simulink model "MPC_Controlled_Booster"  (R2024a)
settings: Solver=VariableStepAuto  StartTime=0  StopTime=1  RelTol=1e-3
values from neighbouring files (symbols this model uses):
  C = (Ioutmax * (1 - (Vin / Vref))) / (fs * delvout)    (= 0.00434027777778)    [RLC_For_MPC.m]
  L = (Vin * (Vref - Vin)) / (delIL * fs * Vref)    (= 0.00144)    [RLC_For_MPC.m]
  R = Vref / Ioutmax    (= 1.152)    [RLC_For_MPC.m]
  Vin = 12    [RLC_For_MPC.m]
libraries: spsSeriesRLCBranchLib x3, spsCurrentMeasurementLib x2, spsVoltageMeasurementLib x2, spsDCVoltageSourceLib x1, spsDiodeLib x1, spsIGBTLib x1, spsPWMGeneratorDCDCLib x1, sps_lib x1
settings Model: Creator=Razowan  LastModifiedBy=Razowan
settings DataIOCC: ReturnWorkspaceOutputs=off

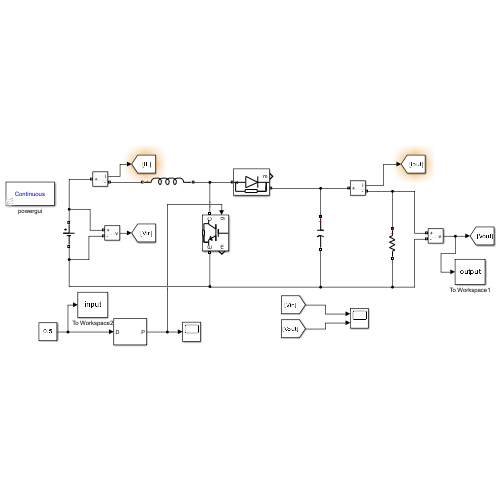
[thumbnail: Simulink's stored preview of the top-level diagram]
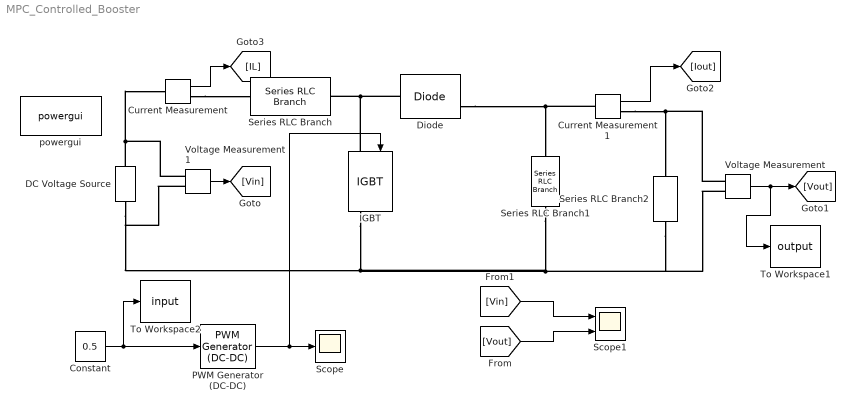
== system MPC_Controlled_Booster ==
  Constant : Constant  Value=0.5
  Current Measurement : spsCurrentMeasurementLib/Current Measurement  PhasorSimulation=off  OutputType=Complex  PSBequivalent=0
  Current Measurement1 : spsCurrentMeasurementLib/Current Measurement  PhasorSimulation=off  OutputType=Complex  PSBequivalent=0
  DC Voltage Source : spsDCVoltageSourceLib/DC Voltage Source  Amplitude=Vin  Measurements=None
  Diode : spsDiodeLib/Diode  Ron=0.001  Lon=0  Vf=0.8  IC=0  UseSnubber=0  Rs=500  Cs=250e-9  Measurements=on
  IGBT : spsIGBTLib/IGBT  Ron=0.001  Lon=0  Vf=1  Tf=1e-6  Tt=2e-6  IC=0  Rs=1e5  Cs=inf  Measurements=on
  PWM Generator (DC-DC) : spsPWMGeneratorDCDCLib/PWM Generator (DC-DC)  Fsw=10000  Ts=0
  Scope : Scope
  Scope1 : Scope  NumInputPorts=2
  Series RLC Branch : spsSeriesRLCBranchLib/Series RLC Branch  LConnTagsString=__new0  RConnTagsString=__new0  BranchType=L  Resistance=1  Inductance=L  SetiL0=off  InitialCurrent=0  Capacitance=1e-6  Setx0=off  InitialVoltage=0  Measurements=None
  Series RLC Branch1 : spsSeriesRLCBranchLib/Series RLC Branch  LConnTagsString=__new0  RConnTagsString=__new0  BranchType=C  Resistance=1  Inductance=L  SetiL0=off  InitialCurrent=0  Capacitance=C  Setx0=off  InitialVoltage=0  Measurements=None
  Series RLC Branch2 : spsSeriesRLCBranchLib/Series RLC Branch  LConnTagsString=__new0  RConnTagsString=__new0  BranchType=R  Resistance=R  Inductance=L  SetiL0=off  InitialCurrent=0  Capacitance=1e-6  Setx0=off  InitialVoltage=0  Measurements=None
  To Workspace1 : ToWorkspace  VariableName=output  SampleTime=0.00001
      settings: Save2DSignal=2-D array (concatenate along first dimension)
  To Workspace2 : ToWorkspace  VariableName=input  SampleTime=0.00001
      settings: Save2DSignal=2-D array (concatenate along first dimension)
  Voltage Measurement : spsVoltageMeasurementLib/Voltage Measurement  PhasorSimulation=off  OutputType=Complex  PSBequivalent=0
  Voltage Measurement1 : spsVoltageMeasurementLib/Voltage Measurement  PhasorSimulation=off  OutputType=Complex  PSBequivalent=0
  powergui : sps_lib/powergui  Priority=1  SimulationMode=Continuous  SampleTime=1e-6  frequency=60  Iterations=50  frequencyindice=0  Pbase=100e6  ErrMax=1e-4  UnitsV=kV  UnitsW=MW  buscounter=0  FunctionMessages=off  echomessages=off  EnableUseOfTLC=off  CurrentSourceSwitches=off  DisableSnubberDevices=off  DisableRonSwitches=off  DisableVfSwitches=off  DisplayEquations=off  AutomaticDiscreteSolvers=off  SolverType=Tustin/Backward Euler (TBE)  Interpol=off  ExternalGateDelay=off  methode=off  Ts=100  x0status=blocks  SPID=on  SwTol=0  HookPort=off  NonlinearTolerance=1e-4  nMaxIteration=100  ContinueOnMaxIteration=off  RestoreLinks=warning  ResistiveCurrentMeasurement=off  Frange=[0:2:500]  Ylog=off  Xlog=on  ShowGrid=off  save=off  variable=ZData  structure=0  ZoomFFT=off  StartTime=0.0  cycles=1  DisplayStyle=1  fundamental=60  FreqAxis=off  MaxFrequency=1000  frequencyindicesteady=1  RmsSteady=1  display=off
  wires:
  Voltage Measurement1/1 -> [Vin]
  Current Measurement/1 -> [IL]
  Current Measurement1/1 -> [Iout]
  Constant/1 -> To Workspace2/1, PWM Generator (DC-DC)/1
  PWM Generator (DC-DC)/1 -> Scope/1, IGBT/1
  [Vout] -> Scope1/2
  [Vin] -> Scope1/1
  Voltage Measurement/1 -> To Workspace1/1, [Vout]
  connections:
  Current Measurement/RConn1 -- Series RLC Branch/LConn1
  Voltage Measurement1/LConn1 -- DC Voltage Source/RConn1 -- Current Measurement/LConn1
  Diode/LConn1 -- IGBT/LConn1 -- Series RLC Branch/RConn1
  IGBT/RConn1 -- DC Voltage Source/LConn1 -- Voltage Measurement1/LConn2 -- Voltage Measurement/LConn2 -- Series RLC Branch2/RConn1 -- Series RLC Branch1/RConn1
  Diode/RConn1 -- Current Measurement1/LConn1 -- Series RLC Branch1/LConn1
  Voltage Measurement/LConn1 -- Current Measurement1/RConn1 -- Series RLC Branch2/LConn1
